simulink model "Simulasi_3DOFLengkap5"  (R2024b)
settings: Solver=VariableStepAuto  StartTime=0.0  StopTime=500  FixedStep=au  RelTol=1e-10
undefined symbols (not defined in the file): controller, dr2, dr3, du2, du3, dv2, dv3, gamma, Gpi, guidance, IzMinNrd, m, magnitude, Nr, x_8, x_custom, x_elips, x_ling, x_s, Xu, Xud, y_8, y_custom, y_elips, y_ling, y_s, Yv, Yvd
libraries: fuzblock x7, simulink x6, mssSimulink x1
(part 2 of 2)

== matlab function Simulasi_3DOFLengkap5/MATLAB Function ==
  settings: updateMethod=DISCRETE
  data: x input; y input
% function realTimePlot(x, y, waypointX, waypointY)
% %#codegen
% coder.extrinsic('figure', 'plot', 'hold', 'grid', 'xlabel', 'ylabel', ...
%     'title', 'set', 'drawnow', 'isempty', 'gcf', 'xlim', 'ylim', 'legend');
% 
% % Persistent variables
% persistent xData yData hPlot fig hWaypoint;
% 
% % Inisialisasi variabel pada iterasi pertama
% if isempty(fig)
%     fig = figure('Name', 'Real-Time Plot', 'NumberTitle', 'off');
%     hold on;
%     grid on;
%     xlabel('X');
%     ylabel('Y');
%     title('Real-Time Plot of X vs Y with Waypoints');
%     xData = [];
%     yData = [];
%     hPlot = plot(NaN, NaN, 'b.-', 'MarkerSize', 10); % Plot lintasan
%     hWaypoint = plot(waypointX, waypointY, 'r--', 'MarkerSize', 1, 'LineWidth', 1); % Plot waypoint
%     legend('USV Path', 'Waypoint');
% end
% 
% % Pastikan dimensi konsisten
% if isrow(x)
%     x = x'; % Pastikan x adalah vektor kolom
% end
% if isrow(y)
%     y = y'; % Pastikan y adalah vektor kolom
% end
% 
% % Tambahkan data baru
% if isempty(xData)
%     xData = x; % Inisialisasi xData jika kosong
%     yData = y; % Inisialisasi yData jika kosong
% else
%     xData = [xData; x]; % Tambahkan data baru sebagai baris baru
%     yData = [yData; y]; % Tambahkan data baru sebagai baris baru
% end
% 
% % Perbarui plot lintasan
% set(hPlot, 'XData', xData, 'YData', yData);
% 
% % Perbarui waypoint (jika berubah)
% set(hWaypoint, 'XData', waypointX, 'YData', waypointY);
% % 
% % % Atur batas sumbu secara otomatis jika perlu
% % xlim([min([xData; waypointX]) - 5, max([xData; waypointX]) + 5]);
% % ylim([min([yData; waypointY]) - 5, max([yData; waypointY]) + 5]);
% 
% % Perbarui jendela plot
% drawnow;
% 
% end

function realTimePlot(x, y)
%#codegen
% Fungsi untuk menampilkan plot real-time dari input x dan y
% Input:
%   x - Nilai input x (titik pada sumbu X)
%   y - Nilai input y (titik pada sumbu Y)

% Deklarasikan fungsi grafik sebagai extrinsic
coder.extrinsic('figure', 'plot', 'hold', 'grid', 'xlabel', 'ylabel', ...
    'title', 'set', 'drawnow', 'isempty', 'gcf', 'xlim', 'ylim');

% Persistent variables
persistent xData yData hPlot fig;

% Inisialisasi variabel pada iterasi pertama
if isempty(fig)
    fig = figure('Name', 'Real-Time Plot', 'NumberTitle', 'off');
    hold on;
    grid on;
    xlabel('X');
    ylabel('Y');
    title('Real-Time Plot of X vs Y');
    xData = [];
    yData = [];
    hPlot = plot(NaN, NaN, 'b.-', 'MarkerSize', 10); % Buat plot awal
end

% Tambahkan data baru
xData = [xData, x];
yData = [yData, y];

% Perbarui plot
set(hPlot, 'XData', xData, 'YData', yData);

% Atur batas sumbu secara otomatis jika perlu
xlim([min(xData) - 1, max(xData) + 1]);
ylim([min(yData) - 1, max(yData) + 1]);

% Perbarui jendela plot
drawnow;

end

== matlab function Simulasi_3DOFLengkap5/Backup Tidak Digunakan/Konversi Sinyal 1 ==
  data: Throttle input; Tu output; Tv output; Rudder input; Tr output; Vx input
function [Tu,Tv,Tr] = CV(Throttle,Rudder,Vx)
Kthrust = 0.0201;
Tu= Kthrust*1097.6*(1-exp(-13*abs(Throttle)/100));
Tv=0;
Tr = 18*(6.75*(10^-3)).*1.*Vx.^2.*(Rudder/100);

== matlab function Simulasi_3DOFLengkap5/Subsystem/ALOS Guidance ==
  settings: updateMethod=DISCRETE
  data: x input; psi_d output; y input; Delta input; gamma input; R_switch input; xdata input; ydata input; U input; K_f input; h input; x_e output; y_e output; Gpi input
function [psi_d,x_e,y_e]= fcn(x,y,Delta,gamma,R_switch,xdata,ydata,U,K_f,h,Gpi)

% waypoints
wpt.pos.x = xdata;
wpt.pos.y = ydata;

% ALOS guidance law
[psi_d,x_e,y_e] = ALOSpsi(x,y,Delta,gamma,h,R_switch,wpt,U,K_f,Gpi);

end
